simulink model "ConfiguredHevMmVirtualVehicle"  (R2025b)
settings: configuration reference "VehicleVariable" (kept outside this file)
StartFcn:
  | %tic
StopFcn:
  | %toc
model workspace (MAT data in the model file):
  ExtDrvCmdsSwitch : Simulink.Parameter (value not decoded)
  ExtDrvRefSwitch : Simulink.Parameter (value not decoded)
  ExtEnvSwitch : Simulink.Parameter (value not decoded)
  ExtGndSwitch : Simulink.Parameter (value not decoded)
symbols that are objects in the model workspace (value not decoded): ExtDrvCmdsSwitch, ExtDrvRefSwitch, ExtEnvSwitch, ExtGndSwitch
undefined symbols (not defined in the file or in its folder): AmbTemp, BaroPress, CurvGradRef, CurvRef, DCM, DriverAeroRes, DriverDrivelineRes, DriverInitialGear, DriverPreviewDist, DriverRollRes, DriverShiftTime, DriverTimeConst, DriverTractiveForce, EnvAbsPrs, EnvAirTemp, EnvGrvty, EnvNomFrictionScaling, EnvNominalGrade, EnvScnFrictionMap, EnvScnFrictionMapXBpts, EnvScnFrictionMapYBpts, EnvScnHeightMap, EnvScnHeightMapXBpts, EnvScnHeightMapYBpts, EnvWindVelX, EnvWindVelY, EnvWindVelZ, Gnd, Grade, HazzardCmd, HighBeamCmd, lambda_mux, LeftSignalCmd, LngRef, LowBeamCmd, LtrRef, PhiRef, PlntVehDstCGFrntAxl, PlntVehDstCGRearAxl, PlntVehInitLatPos, PlntVehInitLongPos, PlntVehInitPitchAng, PlntVehInitRollAng, PlntVehInitVertPos, PlntVehInitYawAng, PlntVehMass, PlntVehTrckWdth, PlntVehYawMomentInertia, PlntWhlLdRadiusFrnt, PlntWhlLdRadiusRear, RightSignalCmd, ScnCRRadius, Sim3dSensor, Wind, XRef, YRef, Z
libraries: simulink x28, autolibutils x8, autolibsharedcommon x7, vehdynlibscenariocommon x7, vehdynlibviscommon x4, vehdynlibdriver x2, sim3dgroundtruthsensorlib x2, sim3dlib x2, autolibshared x2, sim3dautolib x2, sl3dlib x1, sharedtransform x1
(part 3 of 6)

== system ConfiguredHevMmVirtualVehicle/Driver Commands/Driver Commands/Longitudinal Driver ==
  VehRef : Inport
  VehFdbk : Inport  Port=2
  Env : Inport  Port=3
  Bus Creator1 : BusCreator  Inputs=6
  Bus Selector1 : BusSelector  OutputSignals=DrvCmd.SteerCmd.SteerCmd,DrvRef.LngRef,DrvCmd.AccelCmd.EnblAccelCmd,DrvCmd.AccelCmd.AccelCmd,DrvCmd.AccelCmd.AccelHld,DrvCmd.AccelCmd.AccelZero,DrvCmd.DecelCmd.EnblDecelCmd,DrvCmd.DecelCmd.DecelCmd,DrvCmd.DecelCmd.DecelHld,DrvCmd.DecelCmd.DecelZero
  Constant : Constant  Value=false
  Hill Hold & Stop : Subsystem
  Longitudinal Driver : Subsystem  SystemSampleTime=.01  mask(Longitudinal Driver){extAccelOvr=on, extDecelOvr=on, extAccelHld=on, extDecelHld=on, extAccelZero=on, extDecelZero=on, cntrlType=Predictive, shftType=Reverse, Neutral, Drive, velUnits=m/s, gearOut=on, Kp=10, Ki=5, Kff=.1, Kg=0, VehVelVec=[0 100], KffVec=[.1 .1], KpVec=[10 10], KiVec=[5 5], KgVec=[0 0], m=PlntVehMass, Kpt=DriverTractiveForce, tau=DriverTimeConst, L=DriverPreviewDist, aR=DriverRollRes, bR=DriverDrivelineRes, cR=DriverAeroRes, g=EnvGrvty, vnom=5, Kaw=1, tauerr=.01, tauPt=2, GearInit=DriverInitialGear, tShift=DriverShiftTime, pdlVec=[0.1 0.4 0.5 0.9], upShftTbl=[-1 12.9375 26.4375 39.9375 51.18749999999999 62.4375 72.84375 83.25;-1 16.3125 29.8125 43.3125 54.5624 65.8125 76.78125 87.75;-1 19.6875 33.1875 46.68749999999999 57.9375 69.1875 80.71875 92.25;-1 33 52.5 77.25 100.5 138.75 161.875 185], dwnShftTbl=[1 9.5625 23.0625 36.5625 47.8125 59.0625 68.90625 78.75;1 12.9375 26.4375 39.9375 51.18749999999999 62.4375 72.84375 83.25;1 16.3125 29.8125 43.3125 54.562499 65.8125 76.78125 87.75;1 19.6875 33.1875 46.68749999999999 57.9375 69.1875 80.71875 92.25], tClutch=.5, tRev=.5, tPark=120, aMode=6, UpGearVec=[0  1  2  3  4  5  6  7], DownGearVec=[1  2  3  4  5  6  7  8]}
      mask prompts: extAccelOvr "autoblks_shared:autoblkLongitudinalDriver:blkPrm_extAccelOvr"; extDecelOvr "autoblks_shared:autoblkLongitudinalDriver:blkPrm_extDeccelOvr"; extAccelHld "autoblks_shared:autoblkLongitudinalDriver:blkPrm_extAccelHld"; extDecelHld "autoblks_shared:autoblkLongitudinalDriver:blkPrm_extDeccelHld"; extAccelZero "autoblks_shared:autoblkLongitudinalDriver:blkPrm_extAccelZero"; extDecelZero "autoblks_shared:autoblkLongitudinalDriver:blkPrm_extDeccelZero"; cntrlType "autoblks_shared:autoblkLongitudinalDriver:blkPrm_cntrlType"; shftType "autoblks_shared:autoblkLongitudinalDriver:blkPrm_shftType"; velUnits "autoblks_shared:autoblkLongitudinalDriver:blkPrm_velUnits"; gearOut "autoblks_shared:autoblkLongitudinalDriver:blkPrm_gearOut"; Kp "autoblks_shared:autoblkLongitudinalDriver:blkPrm_Kp"; Ki "autoblks_shared:autoblkLongitudinalDriver:blkPrm_Ki"; Kff "autoblks_shared:autoblkLongitudinalDriver:blkPrm_Kff"; Kg "autoblks_shared:autoblkLongitudinalDriver:blkPrm_Kg"; VehVelVec "autoblks_shared:autoblkLongitudinalDriver:blkPrm_VehVelVec"; KffVec "autoblks_shared:autoblkLongitudinalDriver:blkPrm_KffVec"; KpVec "autoblks_shared:autoblkLongitudinalDriver:blkPrm_KpVec"; KiVec "autoblks_shared:autoblkLongitudinalDriver:blkPrm_KiVec"; KgVec "autoblks_shared:autoblkLongitudinalDriver:blkPrm_KgVec"; m "autoblks_shared:autoblkLongitudinalDriver:blkPrm_m"; Kpt "autoblks_shared:autoblkLongitudinalDriver:blkPrm_Kpt"; tau "autoblks_shared:autoblkLongitudinalDriver:blkPrm_tau"; L "autoblks_shared:autoblkLongitudinalDriver:blkPrm_L"; aR "autoblks_shared:autoblkLongitudinalDriver:blkPrm_aR"; bR "autoblks_shared:autoblkLongitudinalDriver:blkPrm_bR"; cR "autoblks_shared:autoblkLongitudinalDriver:blkPrm_cR"; g "autoblks_shared:autoblkLongitudinalDriver:blkPrm_g"; vnom "autoblks_shared:autoblkLongitudinalDriver:blkPrm_vnom"; Kaw "autoblks_shared:autoblkLongitudinalDriver:blkPrm_Kaw"; tauerr "autoblks_shared:autoblkLongitudinalDriver:blkPrm_tauerr"; tauPt "autoblks_shared:autoblkLongitudinalDriver:blkPrm_tauPt"; GearInit "autoblks_shared:autoblkLongitudinalDriver:blkPrm_GearInit"; tShift "autoblks_shared:autoblkLongitudinalDriver:blkPrm_tShift"; pdlVec "autoblks_shared:autoblkLongitudinalDriver:blkPrm_pdlVec"; upShftTbl "autoblks_shared:autoblkLongitudinalDriver:blkPrm_upShftTbl"; dwnShftTbl "autoblks_shared:autoblkLongitudinalDriver:blkPrm_dwnShftTbl"; tClutch "autoblks_shared:autoblkLongitudinalDriver:blkPrm_tClutch"; tRev "autoblks_shared:autoblkLongitudinalDriver:blkPrm_tRev"; tPark "autoblks_shared:autoblkLongitudinalDriver:blkPrm_tPark"; UpGearVec "autoblks_shared:autoblkLongitudinalDriver:blkPrm_UpGearVec"; DownGearVec "autoblks_shared:autoblkLongitudinalDriver:blkPrm_DownGearVec"
      mask help: autoblks_shared:autoblkLongitudinalDriver:blkDesc
      mask init:
      | [~]=autosharedicon('autoliboperlong',gcb,0);
      mask Help: eval('autosharedhelp(''pbopmodlong'')');
      mask TypeOptions cntrlType: autoblks_shared:autoblkLongitudinalDriver:blkCmb_cntrlType_c1 | autoblks_shared:autoblkLongitudinalDriver:blkCmb_cntrlType_c2 | autoblks_shared:autoblkLongitudinalDriver:blkCmb_cntrlType_c3
      mask Callback cntrlType: [~]=autosharedicon('autoliboperlong',gcb,1);
      mask TypeOptions shftType: Longitudinal Driver/shftType
      mask Callback shftType: [~]=autosharedicon('autoliboperlong',gcb,1);
      mask TypeOptions velUnits: VelRef/Unit
      mask Callback velUnits: [~]=autosharedicon('autoliboperlong',gcb,1);
      mask DialogControl modeConfig Prompt: autoblks_shared:autoblkLongitudinalDriver:blkDlg_modeConfig
      mask DialogControl sigConfigPanel Prompt: autoblks_shared:autoblkLongitudinalDriver:blkDlg_sigConfigPanel
      mask DialogControl extAccelOvr Prompt: Accelerator override
      mask DialogControl extDecelOvr Prompt: Decelerator override
      mask DialogControl extAccelHld Prompt: Accelerator hold
      mask DialogControl extDecelHld Prompt: Decelerator hold
      mask DialogControl extAccelZero Prompt: Accelerator disable
      mask DialogControl extDecelZero Prompt: Decelerator disable
      mask DialogControl cntrlType Prompt: Control type, cntrlType:
      mask DialogControl shftType Prompt: Shift type, shftType:
      mask DialogControl velUnits Prompt: Reference and feedback units, velUnits [velUnits]:
      mask DialogControl gearOut Prompt: Output gear signal
      mask DialogControl CntrlParamPanel Prompt: autoblks_shared:autoblkLongitudinalDriver:blkDlg_CntrlParamPanel
      mask DialogControl PIParam Prompt: autoblks_shared:autoblkLongitudinalDriver:blkDlg_PIParam
      mask DialogControl Kp Prompt: Proportional gain, Kp []:
      mask DialogControl Ki Prompt: Integral gain, Ki []:
      mask DialogControl Kff Prompt: Velocity feed-forward, Kff []:
      mask DialogControl Kg Prompt: Grade angle feed-forward, Kg [1/deg]:
      mask DialogControl PISchedParam Prompt: autoblks_shared:autoblkLongitudinalDriver:blkDlg_PISchedParam
      mask DialogControl VehVelVec Prompt: Velocity gain breakpoints:
      mask DialogControl KffVec Prompt: Velocity feed-forward gain values, KffVec []:
      mask DialogControl KpVec Prompt: Proportional gain values, KpVec []:
      mask DialogControl KiVec Prompt: Integral gain values, KiVec []:
      mask DialogControl KgVec Prompt: Grade angle feed-forward values, KgVec [1/deg]:
      mask DialogControl PredParam Prompt: autoblks_shared:autoblkLongitudinalDriver:blkDlg_PredParam
      mask DialogControl m Prompt: Vehicle mass, m [kg]:
      mask DialogControl Kpt Prompt: Effective vehicle total tractive force, Kpt [N]:
      mask DialogControl tau Prompt: Driver response time, tau [s]:
      mask DialogControl L Prompt: Preview distance, L [m]:
      mask DialogControl aR Prompt: Rolling resistance coefficient, aR [N]:
      mask DialogControl bR Prompt: Rolling and driveline resistance coefficient, bR [N*s/m]:
      mask DialogControl cR Prompt: Aerodynamic drag coefficient, cR [N*s^2/m^2]:
      mask DialogControl g Prompt: Gravitational constant, g [m/s^2]:
      mask DialogControl vnom Prompt: Nominal speed, vnom [velUnits]:
      mask DialogControl Kaw Prompt: Anti-windup, Kaw []:
      mask DialogControl tauerr Prompt: Error filter time constant, tauerr [s]:
      mask DialogControl tauPt Prompt: Powertrain time constant, tauPt [s]:
      mask DialogControl shiftParamPanel Prompt: autoblks_shared:autoblkLongitudinalDriver:blkDlg_shiftParamPanel
      mask DialogControl GearInit Prompt: Initial gear, GearInit []:
      mask DialogControl tShift Prompt: Time required to shift, tShift [s]:
      mask DialogControl pdlVec Prompt: Up and down shift accelerator pedal positions, pdlVec []:
      mask DialogControl upShftTbl Prompt: Upshift velocity data table, upShftTbl [velUnits]:
      mask DialogControl dwnShftTbl Prompt: Downshift velocity data table, dwnShftTbl [velUnits]:
      mask DialogControl tClutch Prompt: Time required to shift, tClutch [s]:
      mask DialogControl tRev Prompt: Time required to engage reverse from neutral, tRev [s]:
      mask DialogControl tPark Prompt: Time required to engage park from neutral, tPark [s]:
      mask DialogControl UpGearVec Prompt: Upshift gear vector, UpGearVec []:
      mask DialogControl DownGearVec Prompt: Downshift gear vector, DownGearVec []:
      mask Display:
      | try
      |     IconInfo = autosharedicon('autoliboperlong', gcb, 4);
      | 
      |     image(IconInfo.image, IconInfo.position);
      | 
      |     for i = 1:numel(IconInfo.lconn)
      |         port_label('lconn', i, IconInfo.lconn{i})
      |     end
      | 
      |     for j = 1:numel(IconInfo.rconn)
      |         port_label('rconn', j, IconInfo.rconn{j})
      |     end
      | 
      |     for k = 1:numel(IconInfo.input)
      |         port_label('input', k, IconInfo.input{k})
      |     end
      | 
      |     for m = 1:numel(IconInfo.output)
      |         port_label('output', m, IconInfo.output{m})
      |     end
      | catch
      |     fprintf('Longitudinal \n Driver')
      | end
  Signal Specification : SignalSpecification  Unit=rad
  Terminator3 : Terminator
  To Nonvirtual Bus : SignalConversion  ConversionOutput=Virtual bus  OverrideOpt=off
  Unit Conversion : UnitConversion
  Unit Conversion1 : UnitConversion
  VVCLightsCmd : Constant  Value=0  OutDataTypeStr=Bus: VVCLightsCmdBUS  SampleTime=-1
  Driver : Outport  VectorParamsAs1DForOutWhenUnconnected=off
  wires:
  Signal Specification/1 -> Bus Creator1/1  "SteerCmd"
  To Nonvirtual Bus/1 -> Bus Creator1/6  "LightsCmd"
  VVCLightsCmd/1 -> To Nonvirtual Bus/1
  Hill Hold & Stop/6(Grade) -> Longitudinal Driver/11(Grade)
  Hill Hold & Stop/5(VelFdbk) -> Longitudinal Driver/10(VelFdbk)
  Bus Selector1/5 -> Longitudinal Driver/4(AccelHld)  "<AccelHld>"
  Unit Conversion1/1 -> Longitudinal Driver/1(VelRef), Hill Hold & Stop/1(LngRef)
  Hill Hold & Stop/4(DecelZero) -> Longitudinal Driver/9(DecelZero)
  Hill Hold & Stop/3(DecelHld) -> Longitudinal Driver/8(DecelHld)
  Env/1 -> Hill Hold & Stop/6(Env)
  Hill Hold & Stop/1(EnblDecelOvr) -> Longitudinal Driver/6(EnblDecelOvr)
  Hill Hold & Stop/2(DecelOvrCmd) -> Longitudinal Driver/7(DecelOvrCmd)
  Bus Selector1/10 -> Hill Hold & Stop/5(<DecelZero>)  "<DecelZero>"
  Bus Selector1/9 -> Hill Hold & Stop/4(<DecelHld>)  "<DecelHld>"
  Bus Selector1/8 -> Hill Hold & Stop/3(<DecelOvrCmd>)  "<DecelCmd>"
  Bus Selector1/7 -> Hill Hold & Stop/2(<EnblDecelCmd>)  "<EnblDecelCmd>"
  Bus Selector1/6 -> Longitudinal Driver/5(AccelZero)  "<AccelZero>"
  Bus Selector1/4 -> Longitudinal Driver/3(AccelOvrCmd)  "<AccelCmd>"
  Bus Selector1/3 -> Longitudinal Driver/2(EnblAccelOvr)  "<EnblAccelCmd>"
  Constant/1 -> Bus Creator1/5  "IgnSwtch"
  Bus Selector1/1 -> Unit Conversion/1  "<SteerCmd>"
  Longitudinal Driver/4(GearCmd) -> Bus Creator1/4  "GearCmd"
  Longitudinal Driver/2(AccelCmd) -> Bus Creator1/2  "AccelCmd"
  VehFdbk/1 -> Hill Hold & Stop/7(VehFdbk)
  VehRef/1 -> Bus Selector1/1
  Bus Selector1/2 -> Unit Conversion1/1  "<LngRef>"
  Longitudinal Driver/1(Info) -> Terminator3/1
  Longitudinal Driver/3(DecelCmd) -> Bus Creator1/3  "DecelCmd"
  Unit Conversion/1 -> Signal Specification/1
  Bus Creator1/1 -> Driver/1

== system ConfiguredHevMmVirtualVehicle/Driver Commands/Driver Commands/No Driver ==
  VehRef : Inport
  VehFdbk : Inport  Port=2
  Env : Inport  Port=3
  Bus Creator1 : BusCreator  Inputs=6
  Bus Selector1 : BusSelector  OutputSignals=DrvCmd.SteerCmd.SteerCmd,DrvCmd.AccelCmd.AccelCmd,DrvCmd.DecelCmd.DecelCmd,DrvCmd.TransCmd.GearCmd,DrvCmd.IgnModeCmd,DrvCmd.LightsCmd
  Data Type Conversion : DataTypeConversion  SaturateOnIntegerOverflow=off  RndMeth=Floor
  Data Type Conversion1 : DataTypeConversion  SaturateOnIntegerOverflow=off  RndMeth=Floor
  Signal Specification{,1..3} (4 alike) : SignalSpecification  Unit=1
  Signal Specification4 : SignalSpecification  Unit=rad
  Terminator : Terminator
  Terminator1 : Terminator
  To Nonvirtual Bus : SignalConversion  ConversionOutput=Virtual bus  OverrideOpt=off
  Unit Conversion{,1..3} (4 alike) : UnitConversion
  Driver : Outport  VectorParamsAs1DForOutWhenUnconnected=off
  wires:
  Unit Conversion/1 -> Signal Specification4/1
  Data Type Conversion/1 -> Signal Specification3/1
  Unit Conversion3/1 -> Signal Specification2/1
  Unit Conversion2/1 -> Signal Specification1/1
  Unit Conversion1/1 -> Signal Specification/1
  Data Type Conversion1/1 -> Unit Conversion3/1
  Bus Selector1/5 -> Data Type Conversion/1  "<IgnModeCmd>"
  Bus Selector1/6 -> To Nonvirtual Bus/1  "<LightsCmd>"
  Bus Selector1/4 -> Data Type Conversion1/1  "<GearCmd>"
  Bus Selector1/3 -> Unit Conversion2/1  "<DecelCmd>"
  To Nonvirtual Bus/1 -> Bus Creator1/6  "LightsCmd"
  Env/1 -> Terminator1/1
  Signal Specification3/1 -> Bus Creator1/5  "IgnSwtch"
  Bus Selector1/1 -> Unit Conversion/1  "<SteerCmd>"
  Signal Specification2/1 -> Bus Creator1/4  "GearCmd"
  Signal Specification/1 -> Bus Creator1/2  "AccelCmd"
  VehFdbk/1 -> Terminator/1
  VehRef/1 -> Bus Selector1/1
  Bus Selector1/2 -> Unit Conversion1/1  "<AccelCmd>"
  Signal Specification1/1 -> Bus Creator1/3  "DecelCmd"
  Signal Specification4/1 -> Bus Creator1/1  "SteerCmd"
  Bus Creator1/1 -> Driver/1

== system ConfiguredHevMmVirtualVehicle/Driver Commands/Driver Commands/Open Loop ==
  VehFdbk : Inport
  SteerCmd : Inport  Port=2
  AccelCmd : Inport  Port=3
  BrakeCmd : Inport  Port=4
  GearCmd : Inport  Port=5
  Bus Creator1 : BusCreator  Inputs=6
  Constant : Constant  Value=false
  Signal Specification : SignalSpecification  Unit=1
  Signal Specification1 : SignalSpecification  Unit=1
  Signal Specification2 : SignalSpecification  Unit=1
  Terminator : Terminator
  To Nonvirtual Bus : SignalConversion  ConversionOutput=Virtual bus  OverrideOpt=off
  Unit Conversion : UnitConversion
  VVCLightsCmd : Constant  Value=0  OutDataTypeStr=Bus: VVCLightsCmdBUS  SampleTime=-1
  Wheel Angle Limit * Steer Ratio : Gain  Gain=40*pi/180*18
  Driver : Outport  VectorParamsAs1DForOutWhenUnconnected=off
  wires:
  To Nonvirtual Bus/1 -> Bus Creator1/6  "LightsCmd"
  VVCLightsCmd/1 -> To Nonvirtual Bus/1
  Constant/1 -> Bus Creator1/5  "IgnSwtch"
  Signal Specification1/1 -> Bus Creator1/3  "DecelCmd"
  GearCmd/1 -> Signal Specification2/1
  Signal Specification/1 -> Bus Creator1/2  "AccelCmd"
  SteerCmd/1 -> Unit Conversion/1
  VehFdbk/1 -> Terminator/1
  AccelCmd/1 -> Signal Specification/1
  Unit Conversion/1 -> Wheel Angle Limit * Steer Ratio/1
  Bus Creator1/1 -> Driver/1
  Wheel Angle Limit * Steer Ratio/1 -> Bus Creator1/1  "SteerCmd"
  BrakeCmd/1 -> Signal Specification1/1
  Signal Specification2/1 -> Bus Creator1/4  "GearCmd"

== system ConfiguredHevMmVirtualVehicle/Driver Commands/Driver Commands/Predictive Driver ==
  VehRef : Inport
  VehFdbk : Inport  Port=2
  Env : Inport  Port=3
  Bus Creator1 : BusCreator  Inputs=6
  Bus Selector : BusSelector  OutputSignals=Body.InertFrm.Cg.Disp.Y,Body.InertFrm.Cg.Vel.Ydot,Body.InertFrm.Cg.Ang.psi,Body.BdyFrm.Cg.AngVel.r
  Bus Selector1 : BusSelector  OutputSignals=DrvRef.LngRef,DrvRef.LtrRef,DrvCmd.SteerCmd.EnblSteerCmd,DrvCmd.SteerCmd.SteerCmd,DrvCmd.SteerCmd.SteerHld,DrvCmd.SteerCmd.SteerZero,DrvCmd.AccelCmd.EnblAccelCmd,DrvCmd.AccelCmd.AccelCmd,DrvCmd.AccelCmd.AccelHld,DrvCmd.AccelCmd.AccelZero,DrvCmd.DecelCmd.EnblDecelCmd,DrvCmd.DecelCmd.DecelCmd,DrvCmd.DecelCmd.DecelHld,DrvCmd.DecelCmd.DecelZero
  Constant : Constant  Value=false
  Hill Hold & Stop : Subsystem
  Linear Predictive Driver : vehdynlibdriver/Predictive Driver  extAccelOvr=on  extDecelOvr=on  extAccelHld=on  extDecelHld=on  extAccelZero=on  extDecelZero=on  extSteerOvr=on  extSteerHld=on  extSteerZero=on  cntrlType=Predictive  cntrlTypeLat=Predictive  shftType=Reverse, Neutral, Drive  coordMode=SAE J670 (Z-down)  refType=Reference pose  velUnits=m/s  angUnits=rad  gearOut=on  steerOut=on  Kp=3  Ki=1  Kff=1  Kg=0  VehVelVec=[0 100]  KffVec=[.1 .1]  KpVec=[10 10]  KiVec=[5 5]  KgVec=[0 0]  vnom=5  Kaw=1  tauerr=.075  tau=DriverTimeConst  L=DriverPreviewDist  Kpt=DriverTractiveForce  aR=DriverRollRes  bR=DriverDrivelineRes  cR=DriverAeroRes  g=EnvGrvty  vecPose=off  dynamMode=off  PositionGainF=2.5  PositionGainR=2.5  YawRateGain=.2  DelayGain=.2  enableDrift=off  BetaRef=10  KpBeta=1  KpDrift=1  KdDrift=1  KpPsi=1  KOmega=.1  tOmega=.1  a=PlntVehDstCGFrntAxl  b=PlntVehDstCGRearAxl  m=PlntVehMass  Cy_f=DriverFrontCornerStiff  Cy_r=DriverRearCornerStiff  I=PlntVehYawMomentInertia  Ksteer=PlntSteerRatio  theta=DriverWheelRange  Idl=1  Re=PlntWhlLdRadius  lambda_mu=1  GearInit=DriverInitialGear  tShift=DriverShiftTime  pdlVec=[0.1 0.4 0.5 0.9]  upShftTbl=[-1 12.9375 26.4375 39.9375 51.18749999999999 62.4375 72.84375 83.25;-1 16.3125 29.8125 43.3125 54.5624 65.8125 76.78125 87.75;-1 19.6875 33.1875 46.68749999999999 57.9375 69.1875 80.71875 92.25;-1 33 52.5 77.25 100.5 138.75 161.875 185]  dwnShftTbl=[-1 12.9375 26.4375 39.9375 51.18749999999999 62.4375 72.84375 83.25;-1 16.3125 29.8125 43.3125 54.5624 65.8125 76.78125 87.75;-1 19.6875 33.1875 46.68749999999999 57.9375 69.1875 80.71875 92.25;-1 33 52.5 77.25 100.5 138.75 161.875 185]  tClutch=.5  tRev=.5  tPark=120  UpGearVec="[0  1  2  3  4  5  6  7]"  DownGearVec="[1  2  3  4  5  6  7  8]"  aMode=2
  Terminator : Terminator
  To Nonvirtual Bus : SignalConversion  ConversionOutput=Virtual bus  OverrideOpt=off
  Unit Conversion : UnitConversion
  VVCLightsCmd : Constant  Value=0  OutDataTypeStr=Bus: VVCLightsCmdBUS  SampleTime=-1
  Driver : Outport  VectorParamsAs1DForOutWhenUnconnected=off
  wires:
  Bus Selector1/14 -> Hill Hold & Stop/5(<DecelZero>)  "<DecelZero>"
  To Nonvirtual Bus/1 -> Bus Creator1/6  "LightsCmd"
  VVCLightsCmd/1 -> To Nonvirtual Bus/1
  Unit Conversion/1 -> Linear Predictive Driver/1, Hill Hold & Stop/1(LngRef)
  Hill Hold & Stop/1(EnblDecelOvr) -> Linear Predictive Driver/11
  Hill Hold & Stop/2(DecelOvrCmd) -> Linear Predictive Driver/12
  Hill Hold & Stop/3(DecelHld) -> Linear Predictive Driver/13
  Hill Hold & Stop/4(DecelZero) -> Linear Predictive Driver/14
  Hill Hold & Stop/6(VelFdbk) -> Linear Predictive Driver/16
  Hill Hold & Stop/5(Grade) -> Linear Predictive Driver/15
  Env/1 -> Hill Hold & Stop/6(Env)
  Bus Selector1/13 -> Hill Hold & Stop/4(<DecelHld>)  "<DecelHld>"
  Bus Selector1/12 -> Hill Hold & Stop/3(<DecelOvrCmd>)  "<DecelCmd>"
  Bus Selector1/11 -> Hill Hold & Stop/2(<EnblDecelCmd>)  "<EnblDecelCmd>"
  Bus Selector1/9 -> Linear Predictive Driver/9  "<AccelHld>"
  Bus Selector1/8 -> Linear Predictive Driver/8  "<AccelCmd>"
  Bus Selector1/7 -> Linear Predictive Driver/7  "<EnblAccelCmd>"
  Bus Selector1/6 -> Linear Predictive Driver/6  "<SteerZero>"
  Bus Selector1/5 -> Linear Predictive Driver/5  "<SteerHld>"
  Bus Selector1/4 -> Linear Predictive Driver/4  "<SteerCmd>"
  Bus Selector1/3 -> Linear Predictive Driver/3  "<EnblSteerCmd>"
  Constant/1 -> Bus Creator1/5  "IgnSwtch"
  Linear Predictive Driver/5 -> Bus Creator1/4  "GearCmd"
  Linear Predictive Driver/4 -> Bus Creator1/3  "DecelCmd"
  Linear Predictive Driver/2 -> Bus Creator1/1  "SteerCmd"
  Bus Selector1/1 -> Unit Conversion/1  "<LngRef>"
  VehRef/1 -> Bus Selector1/1
  Bus Selector/4 -> Linear Predictive Driver/20  "<r>"
  Bus Selector1/2 -> Linear Predictive Driver/2  "<LtrRef>"
  VehFdbk/1 -> Bus Selector/1, Hill Hold & Stop/7(VehFdbk)
  Bus Selector/3 -> Linear Predictive Driver/19  "<psi>"
  Linear Predictive Driver/1 -> Terminator/1
  Bus Creator1/1 -> Driver/1
  Bus Selector1/10 -> Linear Predictive Driver/10  "<AccelZero>"
  Bus Selector/1 -> Linear Predictive Driver/17  "<Y>"
  Linear Predictive Driver/3 -> Bus Creator1/2  "AccelCmd"
  Bus Selector/2 -> Linear Predictive Driver/18  "<Ydot>"

== system ConfiguredHevMmVirtualVehicle/Driver Commands/Driver Commands/Predictive Stanley Driver ==
  VehRef : Inport
  VehFdbk : Inport  Port=2
  Env : Inport  Port=3
  Bus Creator1 : BusCreator  Inputs=6
  Bus Selector : BusSelector  OutputSignals=Body.InertFrm.Cg.Disp.X,Body.InertFrm.Cg.Disp.Y,Body.InertFrm.Cg.Ang.psi,Body.BdyFrm.Cg.AngVel.r
  Bus Selector1 : BusSelector  OutputSignals=DrvRef.LngRef,DrvRef.XRef,DrvRef.YRef,DrvRef.PhiRef,DrvCmd.SteerCmd.EnblSteerCmd,DrvCmd.SteerCmd.SteerCmd,DrvCmd.SteerCmd.SteerHld,DrvCmd.SteerCmd.SteerZero,DrvCmd.AccelCmd.EnblAccelCmd,DrvCmd.AccelCmd.AccelCmd,DrvCmd.AccelCmd.AccelHld,DrvCmd.AccelCmd.AccelZero,DrvCmd.DecelCmd.EnblDecelCmd,DrvCmd.DecelCmd.DecelCmd,DrvCmd.DecelCmd.DecelHld,DrvCmd.DecelCmd.DecelZero,DrvRef.CurvRef
  Constant : Constant  Value=false
  Hill Hold & Stop : Subsystem
  Linear Predictive Driver : vehdynlibdriver/Predictive Driver  extAccelOvr=on  extDecelOvr=on  extAccelHld=on  extDecelHld=on  extAccelZero=on  extDecelZero=on  extSteerOvr=on  extSteerHld=on  extSteerZero=on  cntrlType=Predictive  cntrlTypeLat=Stanley  shftType=Reverse, Neutral, Drive  coordMode=SAE J670 (Z-down)  refType=Reference pose  velUnits=m/s  angUnits=rad  gearOut=on  steerOut=on  Kp=3  Ki=1  Kff=1  Kg=0  VehVelVec=[0 100]  KffVec=[.1 .1]  KpVec=[10 10]  KiVec=[5 5]  KgVec=[0 0]  vnom=5  Kaw=1  tauerr=.075  tau=DriverTimeConst  L=DriverPreviewDist  Kpt=DriverTractiveForce  aR=DriverRollRes  bR=DriverDrivelineRes  cR=DriverAeroRes  g=EnvGrvty  vecPose=off  dynamMode=on  PositionGainF=DriverPositionGainF  PositionGainR=DriverPositionGainR  YawRateGain=DriverYawRateGain  DelayGain=DriverDelayGain  enableDrift=off  BetaRef=10  KpBeta=1  KpDrift=1  KdDrift=1  KpPsi=1  KOmega=.1  tOmega=.1  a=PlntVehDstCGFrntAxl  b=PlntVehDstCGRearAxl  m=PlntVehMass  Cy_f=DriverFrontCornerStiff  Cy_r=DriverRearCornerStiff  I=PlntVehYawMomentInertia  Ksteer=PlntSteerRatio  theta=DriverWheelRange  Idl=1  Re=PlntWhlLdRadius  lambda_mu=1  GearInit=DriverInitialGear  tShift=DriverShiftTime  pdlVec=[0.1 0.4 0.5 0.9]  upShftTbl=[-1 12.9375 26.4375 39.9375 51.18749999999999 62.4375 72.84375 83.25;-1 16.3125 29.8125 43.3125 54.5624 65.8125 76.78125 87.75;-1 19.6875 33.1875 46.68749999999999 57.9375 69.1875 80.71875 92.25;-1 33 52.5 77.25 100.5 138.75 161.875 185]  dwnShftTbl=[-1 12.9375 26.4375 39.9375 51.18749999999999 62.4375 72.84375 83.25;-1 16.3125 29.8125 43.3125 54.5624 65.8125 76.78125 87.75;-1 19.6875 33.1875 46.68749999999999 57.9375 69.1875 80.71875 92.25;-1 33 52.5 77.25 100.5 138.75 161.875 185]  tClutch=.5  tRev=.5  tPark=120  UpGearVec="[0  1  2  3  4  5  6  7]"  DownGearVec="[1  2  3  4  5  6  7  8]"  aMode=2
  Terminator : Terminator
  To Nonvirtual Bus : SignalConversion  ConversionOutput=Virtual bus  OverrideOpt=off
  Unit Conversion : UnitConversion
  VVCLightsCmd : Constant  Value=0  OutDataTypeStr=Bus: VVCLightsCmdBUS  SampleTime=-1
  Driver : Outport  VectorParamsAs1DForOutWhenUnconnected=off
  wires:
  Bus Selector1/13 -> Hill Hold & Stop/2(<EnblDecelCmd>)  "<EnblDecelCmd>"
  Bus Selector1/14 -> Hill Hold & Stop/3(<DecelOvrCmd>)  "<DecelCmd>"
  Bus Selector1/15 -> Hill Hold & Stop/4(<DecelHld>)  "<DecelHld>"
  Bus Selector1/16 -> Hill Hold & Stop/5(<DecelZero>)  "<DecelZero>"
  Bus Selector1/17 -> Hill Hold & Stop/6(<CurvRef>)  "<CurvRef>"
  Bus Selector1/12 -> Linear Predictive Driver/12  "<AccelZero>"
  Bus Selector/1 -> Linear Predictive Driver/20  "<X>"
  Bus Selector/2 -> Linear Predictive Driver/21  "<Y>"
  Bus Selector/3 -> Linear Predictive Driver/22  "<psi>"
  Bus Selector1/2 -> Linear Predictive Driver/2  "<XRef>"
  Bus Selector1/3 -> Linear Predictive Driver/3  "<YRef>"
  Bus Selector1/4 -> Linear Predictive Driver/4  "<PhiRef>"
  Bus Selector1/5 -> Linear Predictive Driver/5  "<EnblSteerCmd>"
  Bus Selector1/10 -> Linear Predictive Driver/10  "<AccelCmd>"
  Bus Selector1/6 -> Linear Predictive Driver/6  "<SteerCmd>"
  Bus Selector1/9 -> Linear Predictive Driver/9  "<EnblAccelCmd>"
  Bus Selector1/7 -> Linear Predictive Driver/7  "<SteerHld>"
  Bus Selector1/8 -> Linear Predictive Driver/8  "<SteerZero>"
  To Nonvirtual Bus/1 -> Bus Creator1/6  "LightsCmd"
  VVCLightsCmd/1 -> To Nonvirtual Bus/1
  Hill Hold & Stop/6(CurvRef) -> Linear Predictive Driver/18
  Hill Hold & Stop/5(Grade) -> Linear Predictive Driver/17
  Bus Selector/4 -> Linear Predictive Driver/23  "<r>"
  Linear Predictive Driver/3 -> Bus Creator1/2  "AccelCmd"
  Bus Creator1/1 -> Driver/1
  Linear Predictive Driver/1 -> Terminator/1
  VehFdbk/1 -> Bus Selector/1, Hill Hold & Stop/8(VehFdbk)
  VehRef/1 -> Bus Selector1/1
  Bus Selector1/1 -> Unit Conversion/1  "<LngRef>"
  Linear Predictive Driver/2 -> Bus Creator1/1  "SteerCmd"
  Linear Predictive Driver/4 -> Bus Creator1/3  "DecelCmd"
  Linear Predictive Driver/5 -> Bus Creator1/4  "GearCmd"
  Constant/1 -> Bus Creator1/5  "IgnSwtch"
  Bus Selector1/11 -> Linear Predictive Driver/11  "<AccelHld>"
  Env/1 -> Hill Hold & Stop/7(Env)
  Hill Hold & Stop/7(VelFdbk) -> Linear Predictive Driver/19
  Hill Hold & Stop/4(DecelZero) -> Linear Predictive Driver/16
  Hill Hold & Stop/3(DecelHld) -> Linear Predictive Driver/15
  Hill Hold & Stop/2(DecelOvrCmd) -> Linear Predictive Driver/14
  Hill Hold & Stop/1(EnblDecelOvr) -> Linear Predictive Driver/13
  Unit Conversion/1 -> Linear Predictive Driver/1, Hill Hold & Stop/1(LngRef)

== system ConfiguredHevMmVirtualVehicle/Environment/Ground Feedback/3D Engine ==
  WheelFdbk : Inport
  3D Engine Source : Subsystem  Variant=on  VariantControl=Choice  mask(Terrain Source){terrType=Single point}
      mask prompts: terrType "Terrain feedback type:"
      mask help:
      | This variant subsystem provides the option for:
      | - a single point of contact for each wheel with minimal post-processing ideal for smooth surfaces and maximum run-time performance.
      | - multiple points of contact per wheel which may be used when interested in non-smooth terrain at a higher computational cost and requires Vehicle Dynamics Blockset.
      mask TypeOptions terrType: Single point | Multiple points
  Z : Outport  VectorParamsAs1DForOutWhenUnconnected=off
  DCM : Outport  Port=2  VectorParamsAs1DForOutWhenUnconnected=off
  wires:
  WheelFdbk/1 -> 3D Engine Source/1(WheelFdbk)
  3D Engine Source/1(z) -> Z/1
  3D Engine Source/2(DCM) -> DCM/1

== system ConfiguredHevMmVirtualVehicle/Environment/Ground Feedback/Constant ==
  Bus Creator : BusCreator  Inputs=4
  Constant1 : Constant  Value=zeros(4,1)
  Constant2 : Constant  Value=repmat(eye(3),1,1,4)  SampleTime=-1
  Demux : Demux
  Signal Specification : SignalSpecification  Unit=m
  Z : Outport  VectorParamsAs1DForOutWhenUnconnected=off
  DCM : Outport  Port=2  VectorParamsAs1DForOutWhenUnconnected=off
  wires:
  Constant1/1 -> Signal Specification/1
  Signal Specification/1 -> Demux/1
  Demux/4 -> Bus Creator/4  "G_RR_z"
  Demux/1 -> Bus Creator/1  "G_FL_z"
  Demux/3 -> Bus Creator/3  "G_RL_z"
  Demux/2 -> Bus Creator/2  "G_FR_z"
  Bus Creator/1 -> Z/1  "z"
  Constant2/1 -> DCM/1  "DCM"

== system ConfiguredHevMmVirtualVehicle/Environment/Ground Feedback/Height Map ==
  InertFrm : Inport
  "2D Lookup Tbl for Elevation, Z" : Subsystem  TreatAsAtomicUnit=on
      mask init:
      | [~]=vehdynicon('vehdynblk',gcb);
  Bus Creator : BusCreator  Inputs=4
  Bus Selector : BusSelector  OutputSignals=FrntAxl.Lft.Disp.X,FrntAxl.Rght.Disp.X,RearAxl.Lft.Disp.X,RearAxl.Rght.Disp.X
  Bus Selector1 : BusSelector  OutputSignals=FrntAxl.Lft.Disp.Y,FrntAxl.Rght.Disp.Y,RearAxl.Lft.Disp.Y,RearAxl.Rght.Disp.Y
  Constant2 : Constant  Value=repmat(eye(3),1,1,4)  SampleTime=-1
  Demux : Demux
  Signal Specification : SignalSpecification  Unit=m
  Wheel Coordinates : Subsystem
  Z : Outport
  DCM : Outport  Port=2
  wires:
  "2D Lookup Tbl for Elevation, Z"/1(Z) -> Signal Specification/1
  Bus Selector1/4 -> Wheel Coordinates/8(RearAxlRghtY)  "<Y>"
  Bus Selector1/3 -> Wheel Coordinates/7(RearAxlLftY)  "<Y>"
  Bus Selector/1 -> Wheel Coordinates/1(FrntAxlLftX)  "<X>"
  Bus Selector/2 -> Wheel Coordinates/2(FrntAxlRghtX)  "<X>"
  Bus Selector1/2 -> Wheel Coordinates/6(FrntAxlRghtY)  "<Y>"
  Bus Selector/4 -> Wheel Coordinates/4(RearAxlRghtX)  "<X>"
  Bus Selector/3 -> Wheel Coordinates/3(RearAxlLftX)  "<X>"
  Bus Selector1/1 -> Wheel Coordinates/5(FrntAxlLftY)  "<Y>"
  Wheel Coordinates/2(YWhl) -> "2D Lookup Tbl for Elevation, Z"/2(YWhl)
  Wheel Coordinates/1(XWhl) -> "2D Lookup Tbl for Elevation, Z"/1(XWhl)
  InertFrm/1 -> Bus Selector1/1, Bus Selector/1
  Demux/2 -> Bus Creator/2  "G_FR_z"
  Demux/1 -> Bus Creator/1  "G_FL_z"
  Demux/4 -> Bus Creator/4  "G_RR_z"
  Demux/3 -> Bus Creator/3  "G_RL_z"
  Bus Creator/1 -> Z/1  "z"
  Signal Specification/1 -> Demux/1
  Constant2/1 -> DCM/1  "DCM"

== system ConfiguredHevMmVirtualVehicle/Environment/Ground Feedback/Ideal Inclined Plane ==
  InertFrm : Inport
  Bus Creator : BusCreator  Inputs=4
  Bus Selector : BusSelector  OutputSignals=FrntAxl.Lft.Disp.X,FrntAxl.Rght.Disp.X,RearAxl.Lft.Disp.X,RearAxl.Rght.Disp.X
  Bus Selector1 : BusSelector  OutputSignals=FrntAxl.Lft.Disp.Y,FrntAxl.Rght.Disp.Y,RearAxl.Lft.Disp.Y,RearAxl.Rght.Disp.Y
  Demux : Demux
  Ideal Inclined Plane : Subsystem  mask(Ideal Plane Elevation Generator){phi_o=0, theta_o=0, Z_o=0, psi_o=-PlntVehInitYawAng, phi_est=0, theta_est=0, Z_est=5, plane3D=off, planeX=200, planeY=200}
      mask prompts: phi_o "Initial plane bank angle (about global X axis) [rad]:"; theta_o "Initial plane pitch angle (about global Y axis)  [rad]:"; Z_o "Initial plane elevation (at [0,0,0]) [m]"; psi_o "Initial vehicle yaw angle (about global Z axis) [rad]:"; phi_est "Estimated initial vehicle roll angle [rad]:"; theta_est "Estimated initial vehicle pitch angle [rad]:"; Z_est "Estimated initial vehicle elevation [m]"; plane3D "Enable 3D visualization of plane. Requires the Simulink 3D Animation and the 3D visualization enabled (in the Visualization subsystem). The Empty Scene is recommended when activated."; planeX "Total plane length (in X dimension) [m]:"; planeY "Total plane width (in Y dimension) [m]:"
      mask help:
      | This block accepts time varying bank and pitch angles for an idealized planar surface centered at the global origin (Z+up).
      | The plane roll or bank angle, phi, is about the X axis and pitch angle, theta (negative grade), is about the Y axis.
      | A static vertical offset, Z_o, is also permited.
      | Based on the initial plane angles and vertical offset and vehicle pose, estimates of the initial vehicle roll and pitch are calculated (in the vehicle Z+ down frame). These values can be optionally used to udpate the sldds.
      | Caution should be used to esnure the input signals and initial parameters are consistent at initialzation time.
      | If Simulink 3D Animation is available, the visualization will also include a planar checkerboard surface (changing the default scene may be desired in the Visualization subsystem).
      mask init:
      | vehdynicon('vehdynlibzplane',gcb,0,[]);
      mask Callback plane3D: vehdynicon('vehdynlibzplane',gcb,1,[]);
      mask DialogControl initParams Prompt: Setup Parameters
      mask DialogControl slddUpdate Prompt: Vehicle Pose Estimates
      mask DialogControl updateSLDD Prompt: Update data dictionary with initial roll, pitch and yaw estimates
      mask DialogControl updateSLDD Callback: vehdynicon('vehdynlibzplane',gcb,2,'VirtualVehicleTemplate.sldd');
      mask DialogControl sim3d Prompt: Visualization Options
  Rate Limiter : RateLimiter  RisingSlewLimit=10  FallingSlewLimit=-10  SampleTimeMode=inherited
  Rate Limiter1 : RateLimiter  RisingSlewLimit=10  FallingSlewLimit=-10  SampleTimeMode=inherited
  Signal Specification : SignalSpecification  Unit=m
  Signal Specification1 : SignalSpecification  Unit=deg
  Signal Specification2 : SignalSpecification  Unit=deg
  Slider : SliderBlock  ScaleMin=-30  ScaleMax=30
  Slider1 : SliderBlock  ScaleMin=-30  ScaleMax=30
  Unit Conversion : UnitConversion
  Unit Conversion1 : UnitConversion
  Vector Concatenate : Concatenate  NumInputs=4  Mode=Multidimensional array  ConcatenateDimension=3
  Wheel Coordinates : Subsystem
  Z+up : UnaryMinus
  phiPlane : Constant  Value=0
  thetaPlane : Constant  Value=0
  Z : Outport
  DCM : Outport  Port=2
  wires:
  Ideal Inclined Plane/2(DCM) -> Vector Concatenate/1, Vector Concatenate/2, Vector Concatenate/4, Vector Concatenate/3  "DCM"
  Signal Specification/1 -> Demux/1
  Bus Creator/1 -> Z/1  "z"
  Demux/3 -> Bus Creator/3  "G_RL_z"
  Demux/4 -> Bus Creator/4  "G_RR_z"
  Demux/1 -> Bus Creator/1  "G_FL_z"
  Demux/2 -> Bus Creator/2  "G_FR_z"
  InertFrm/1 -> Bus Selector/1, Bus Selector1/1
  Wheel Coordinates/1(XWhl) -> Ideal Inclined Plane/1(X)
  Wheel Coordinates/2(YWhl) -> Z+up/1
  Bus Selector1/1 -> Wheel Coordinates/5(FrntAxlLftY)  "<Y>"
  Bus Selector/3 -> Wheel Coordinates/3(RearAxlLftX)  "<X>"
  Bus Selector/4 -> Wheel Coordinates/4(RearAxlRghtX)  "<X>"
  Bus Selector1/2 -> Wheel Coordinates/6(FrntAxlRghtY)  "<Y>"
  Bus Selector/2 -> Wheel Coordinates/2(FrntAxlRghtX)  "<X>"
  Bus Selector/1 -> Wheel Coordinates/1(FrntAxlLftX)  "<X>"
  Bus Selector1/3 -> Wheel Coordinates/7(RearAxlLftY)  "<Y>"
  Bus Selector1/4 -> Wheel Coordinates/8(RearAxlRghtY)  "<Y>"
  phiPlane/1 -> Rate Limiter/1
  Ideal Inclined Plane/1(Z) -> Signal Specification/1
  thetaPlane/1 -> Rate Limiter1/1
  Z+up/1 -> Ideal Inclined Plane/2(Y)
  Signal Specification2/1 -> Unit Conversion1/1
  Signal Specification1/1 -> Unit Conversion/1
  Unit Conversion1/1 -> Ideal Inclined Plane/3(phi)
  Unit Conversion/1 -> Ideal Inclined Plane/4(theta)
  Vector Concatenate/1 -> DCM/1  "DCM"
  Rate Limiter/1 -> Signal Specification2/1
  Rate Limiter1/1 -> Signal Specification1/1

== system ConfiguredHevMmVirtualVehicle/Environment/Ground Feedback/Three-Axle Constant ==
  Bus Creator : BusCreator  Inputs=6
  Constant1 : Constant  Value=zeros(6,1)
  Constant2 : Constant  Value=repmat(eye(3),1,1,6)  SampleTime=-1
  Demux : Demux  Outputs=6
  Signal Specification : SignalSpecification  Unit=m
  Z : Outport  VectorParamsAs1DForOutWhenUnconnected=off
  DCM : Outport  Port=2  VectorParamsAs1DForOutWhenUnconnected=off
  wires:
  Demux/4 -> Bus Creator/4  "G_MR_z"
  Constant2/1 -> DCM/1  "DCM"
  Bus Creator/1 -> Z/1  "z"
  Demux/2 -> Bus Creator/2  "G_FR_z"
  Demux/3 -> Bus Creator/3  "G_ML_z"
  Signal Specification/1 -> Demux/1
  Constant1/1 -> Signal Specification/1
  Demux/6 -> Bus Creator/6  "G_RR_z"
  Demux/5 -> Bus Creator/5  "G_RL_z"
  Demux/1 -> Bus Creator/1  "G_FL_z"

== system ConfiguredHevMmVirtualVehicle/Environment/Subsystem/Estimated Grade ==
  Gnd : Inport
  Atan : Trigonometry  Operator=atan
  Bus Selector : BusSelector  OutputSignals=z  OutputAsBus=on
  Bus to Vector : BusToVector
  Constant Grade : Constant  Value=EnvNominalGrade  SampleTime=-1
  Constant1 : Constant  Value=PlntVehDstCGFrntAxl+PlntVehDstCGRearAxl  SampleTime=-1
  Divide : Product  Inputs=*/
  Gain : Gain  Gain=.5
  Gain1 : Gain  Gain=.5
  Grade Source : ManualSwitch  CurrentSetting=0
  Signal Specification : SignalSpecification  Unit=rad
  Signal Specification1 : SignalSpecification  Unit=deg
  Signal Specification2 : SignalSpecification  Unit=deg
  Subtract : Sum  Inputs=+-
  Sum of Elements : Sum  Inputs=+
  Sum of Elements1 : Sum  Inputs=+
  Unit Conversion : UnitConversion
  Variant Subsystem : Subsystem  Variant=on  VariantControlMode=label  LabelModeActiveChoice=TwoAxle
  Grade : Outport  PortDimensions=1
  wires:
  Divide/1 -> Atan/1
  Bus Selector/1 -> Bus to Vector/1
  Sum of Elements/1 -> Gain/1
  Gain/1 -> Subtract/1
  Sum of Elements1/1 -> Gain1/1
  Signal Specification/1 -> Unit Conversion/1
  Constant1/1 -> Divide/2
  Gain1/1 -> Subtract/2
  Subtract/1 -> Divide/1
  Atan/1 -> Signal Specification/1
  Grade Source/1 -> Grade/1  "Grade"
  Gnd/1 -> Bus Selector/1
  Bus to Vector/1 -> Variant Subsystem/1(Gnd)
  Constant Grade/1 -> Signal Specification2/1
  Signal Specification2/1 -> Grade Source/2
  Unit Conversion/1 -> Signal Specification1/1
  Signal Specification1/1 -> Grade Source/1  "Grade"
  Variant Subsystem/1(F) -> Sum of Elements/1
  Variant Subsystem/2(R) -> Sum of Elements1/1

== system ConfiguredHevMmVirtualVehicle/Environment/Subsystem/Variant Subsystem ==
  note: 1) Add Subsystem or Model blocks as valid variant choices.
      | 2) You cannot connect blocks at this level. At simulation, connectivity is automatically
      | determined, based on the active variant and port name matching.
  InGnd : Inport
  Three-Axle : Subsystem  VariantControl=ThreeAxle
  Two-Axle : Subsystem  VariantControl=TwoAxle
  z : Outport
  <DCM> : Outport  Port=2
  lambda_mux : Outport  Port=3

== system ConfiguredHevMmVirtualVehicle/Environment/Varying Friction/Constant Friction ==
  Friction Scaling : Constant  Value=ones(4,1).*EnvNomFrictionScaling  SampleTime=0
  FricCoeffLambda : Outport
  wires:
  Friction Scaling/1 -> FricCoeffLambda/1

== system ConfiguredHevMmVirtualVehicle/Environment/Varying Friction/Friction Map ==
  InertFrm : Inport
  2D Lookup Tbl for Scaling Fctr (Lambda) : Subsystem  TreatAsAtomicUnit=on
      mask init:
      | [~]=vehdynicon('vehdynblk',gcb);
  Bus Selector : BusSelector  OutputSignals=FrntAxl.Lft.Disp.X,FrntAxl.Rght.Disp.X,RearAxl.Lft.Disp.X,RearAxl.Rght.Disp.X
  Bus Selector1 : BusSelector  OutputSignals=FrntAxl.Lft.Disp.Y,FrntAxl.Rght.Disp.Y,RearAxl.Lft.Disp.Y,RearAxl.Rght.Disp.Y
  Wheel Coordinates : Subsystem
  FricCoeffLambda : Outport
  wires:
  InertFrm/1 -> Bus Selector1/1, Bus Selector/1
  2D Lookup Tbl for Scaling Fctr (Lambda)/1(FricCoeffLambda) -> FricCoeffLambda/1
  Bus Selector1/4 -> Wheel Coordinates/8(RearAxlRghtY)  "<Y>"
  Bus Selector1/3 -> Wheel Coordinates/7(RearAxlLftY)  "<Y>"
  Bus Selector/1 -> Wheel Coordinates/1(FrntAxlLftX)  "<X>"
  Bus Selector/2 -> Wheel Coordinates/2(FrntAxlRghtX)  "<X>"
  Bus Selector1/2 -> Wheel Coordinates/6(FrntAxlRghtY)  "<Y>"
  Bus Selector/4 -> Wheel Coordinates/4(RearAxlRghtX)  "<X>"
  Bus Selector/3 -> Wheel Coordinates/3(RearAxlLftX)  "<X>"
  Bus Selector1/1 -> Wheel Coordinates/5(FrntAxlLftY)  "<Y>"
  Wheel Coordinates/2(YWhl) -> 2D Lookup Tbl for Scaling Fctr (Lambda)/2(YWhl)
  Wheel Coordinates/1(XWhl) -> 2D Lookup Tbl for Scaling Fctr (Lambda)/1(XWhl)

== system ConfiguredHevMmVirtualVehicle/Environment/Varying Friction/Three-Axle Constant Friction ==
  Friction Scaling : Constant  Value=ones(6,1).*EnvNomFrictionScaling  SampleTime=0
  FricCoeffLambda : Outport
  wires:
  Friction Scaling/1 -> FricCoeffLambda/1

== system ConfiguredHevMmVirtualVehicle/Environment/Varying Friction/Varying Friction ==
  InertFrm : Inport
  Cg : Inport  Port=2
  Bus Selector : BusSelector  OutputSignals=FrntAxl.Lft.Disp.X,FrntAxl.Rght.Disp.X,RearAxl.Lft.Disp.X,RearAxl.Rght.Disp.X
  Bus Selector1 : BusSelector  OutputSignals=FrntAxl.Lft.Disp.Y,FrntAxl.Rght.Disp.Y,RearAxl.Lft.Disp.Y,RearAxl.Rght.Disp.Y
  Road Track Friction : Subsystem  mask(Road Track Friction){surface_popup=Split friction coefficient scaling factor, lambda_g=EnvNomFrictionScaling, lambda_r=.6, r_x0=175, r_y0=-100, r_xw=1000, r_yw=500, aMode=2}
      mask prompts: surface_popup "Type of surface:"; lambda_g "Scaling factor for the friction coefficient of ground, lambda_g :"; lambda_r "Scaling factor for the friction coefficient of rectangular surface, lambda_r :"; r_x0 "X coordinate of lower left corner of rectangular surface, r_x0 [m]:"; r_y0 "Y coordinate of lower left corner of rectangular surface, r_y0 [m]:"; r_xw "Rectangular surface width in X direction, r_xw [m]:"; r_yw "Rectangular surface width in Y direction, r_yw [m]:"
      mask init:
      | % Scaling factor for the friction coefficient around the rectangular region
      | mutable = [lambda_g, lambda_g, lambda_g, lambda_g;
      |            lambda_g, lambda_r, lambda_r, lambda_g; 
      |            lambda_g, lambda_r, lambda_r, lambda_g; 
      |            lambda_g, lambda_g, lambda_g, lambda_g ];
      |        
      | 
      | % The step is distance between breakpoint near the boundary of high and
      | % low friction coefficient
      | 
      | step = 0.01 ; 
      | 
      | % In the mask initialization, xbr and ybr breakpoints are with respect to
      | % Body fixed coordinate system. At time t=0, xbr and ybr breakpoints
      | % updates to Earth (Inertial) Fixed coordinate system. The breakpoints for
      | % the lookup table are added via inputs.
      | 
      | xbr = [(r_x0 - step) , (r_x0 + step), (r_x0 + r_xw - step) , (r_x0 + r_xw + step) ];
      | ybr = [(r_y0 - step) , (r_y0 + step), (r_y0 + r_yw - step) , (r_y0 + r_yw + step) ];
      | 
      | 
      | % To check if the created track is split mu or constant mu
      | 
      | surface_popup = get_param(gcb, 'surface_popup');
      | 
      | if strcmp(surface_popup, 'Split friction coefficient scaling factor')
      |     SplitLambdaTrck = 1;
      | elseif strcmp(surface_popup, 'Constant friction coefficient scaling factor')
      |     SplitLambdaTrck = 0;
      | end
      mask Help: eval('vdynblkshelp(''vdynblkstrack'')');
      mask TypeOptions surface_popup: Constant friction coefficient scaling factor | Split friction coefficient scaling factor
      mask Callback surface_popup:
      | surface_popup = get_param(gcb, 'surface_popup');
      | m = Simulink.Mask.get(gcb);
      | 
      | lambda_g = m.getParameter('lambda_g');
      | lambda_r = m.getParameter('lambda_r');
      | r_x0 = m.getParameter('r_x0');
      | r_y0 = m.getParameter('r_y0');
      | r_xw = m.getParameter('r_xw');
      | r_yw = m.getParameter('r_yw');
      | %track_view = m.getParameter('track_view');
      | 
      | 
      | if strcmp(surface_popup, 'Split friction coefficient scaling factor')
      |     lambda_g.Visible = 'on';
      |     lambda_r.Visible = 'on';
      |     r_x0.Visible = 'on';
      |     r_y0.Visible = 'on';
      |     r_xw.Visible = 'on';
      |     r_yw.Visible = 'on';
      |     %track_view.Visible = 'on';
      | 
      | elseif strcmp(surface_popup,'Constant friction coefficient scaling factor')
      |     lambda_g.Visible = 'on';
      |     lambda_r.Visible = 'off';
      |     r_x0.Visible = 'off';
      |     r_y0.Visible = 'off';
      |     r_xw.Visible = 'off';
      |     r_yw.Visible = 'off';
      |     %track_view.Visible = 'off';
      | end
      | [~]=autosharedicon('autolibutils',gcb,0);
      mask DialogControl DescGroupVar Prompt: Track description  (mask)
      mask DialogControl DescTextVar Prompt: Generates a default or user-specified track which creates a rectangular surface of specified friction coefficient. The location of rectangular surface is relative to the origin of Body Fixed Coordinate System.The input of the block is X and Y coordinates of the wheel from the vehicle feedback bus. The block output is friction coefficient for all the wheels.
  Wheel Coordinates : Subsystem
  FricCoeffLambda : Outport
  wires:
  Bus Selector1/1 -> Wheel Coordinates/5(FrntAxlLftY)  "<Y>"
  Bus Selector/3 -> Wheel Coordinates/3(RearAxlLftX)  "<X>"
  Bus Selector/4 -> Wheel Coordinates/4(RearAxlRghtX)  "<X>"
  Wheel Coordinates/1(XWhl) -> Road Track Friction/1(XWhl)
  Bus Selector1/2 -> Wheel Coordinates/6(FrntAxlRghtY)  "<Y>"
  Bus Selector/2 -> Wheel Coordinates/2(FrntAxlRghtX)  "<X>"
  Bus Selector/1 -> Wheel Coordinates/1(FrntAxlLftX)  "<X>"
  Bus Selector1/3 -> Wheel Coordinates/7(RearAxlLftY)  "<Y>"
  Bus Selector1/4 -> Wheel Coordinates/8(RearAxlRghtY)  "<Y>"
  Cg/1 -> Road Track Friction/3(Cg)
  Wheel Coordinates/2(YWhl) -> Road Track Friction/2(YWhl)
  Road Track Friction/1(FricCoeffLambda) -> FricCoeffLambda/1
  InertFrm/1 -> Bus Selector1/1, Bus Selector/1

== system ConfiguredHevMmVirtualVehicle/Scenarios/Coordinate Systems/ISO 8855 (Z-up) ==
  ExtDrvRefIn : Inport
  ExtDrvCmdIn : Inport  Port=2
  Bus Assignment : BusAssignment  AssignedSignals=LtrRef,YRef,PhiRef,CurvRef,CurvGradRef
  Bus Assignment1 : BusAssignment  AssignedSignals=SteerCmd.SteerCmd
  Bus Selector : BusSelector  OutputSignals=LtrRef,YRef,PhiRef,CurvRef,CurvGradRef
  Bus Selector1 : BusSelector  OutputSignals=SteerCmd.SteerCmd
  Unary Minus{,1..5} (6 alike) : UnaryMinus
  ExtDrvRef : Outport
  ExtDrvCmd : Outport  Port=2
  wires:
  ExtDrvRefIn/1 -> Bus Assignment/1, Bus Selector/1
  ExtDrvCmdIn/1 -> Bus Assignment1/1, Bus Selector1/1
  Unary Minus/1 -> Bus Assignment/2
  Bus Assignment1/1 -> ExtDrvCmd/1
  Bus Assignment/1 -> ExtDrvRef/1
  Bus Selector/1 -> Unary Minus/1  "<LtrRef>"
  Unary Minus2/1 -> Bus Assignment/3
  Unary Minus3/1 -> Bus Assignment/4
  Unary Minus4/1 -> Bus Assignment/5
  Unary Minus5/1 -> Bus Assignment/6
  Bus Selector/2 -> Unary Minus2/1  "<YRef>"
  Bus Selector/3 -> Unary Minus3/1  "<PhiRef>"
  Bus Selector/4 -> Unary Minus4/1  "<CurvRef>"
  Bus Selector/5 -> Unary Minus5/1  "<CurvGradRef>"
  Unary Minus1/1 -> Bus Assignment1/2
  Bus Selector1/1 -> Unary Minus1/1  "<SteerCmd>"

== system ConfiguredHevMmVirtualVehicle/Scenarios/Coordinate Systems/SAE J670 (Z-down) ==
  ExtDrvRefIn : Inport
  ExtDrvCmdIn : Inport  Port=2
  ExtDrvRef : Outport
  ExtDrvCmd : Outport  Port=2
  wires:
  ExtDrvCmdIn/1 -> ExtDrvCmd/1
  ExtDrvRefIn/1 -> ExtDrvRef/1

== system ConfiguredHevMmVirtualVehicle/Scenarios/Reference Generator/Braking ==
  "VehFdbk " : Inport
  Braking : vehdynlibscenariocommon/Acceleration and Deceleration Signal Input  tStart=ScnStartTime  ax=ScnBrkAx  velRef=ScnLongVelRef  velRefUnit=mph  brakingType=Longitudinal displacement  tBrake=15  xBrake=ScnBrkXbrake  axDecel=ScnBrkAxdec  steerZero=on  faultTracking=off  bufferSize=4096  velMaxDiff=1  velMeanDiff=2  rMaxDiff=1  steerMaxDiff=3  stopOnFault=off  aMode=2
      settings: LibrarySourceBlock=vehdynlibscenario/Acceleration and Braking
  Bus Creator : BusCreator  Inputs=3
  Bus Selector : BusSelector  OutputSignals=Body.BdyFrm.Cg.Vel.xdot
  Constant : Constant  Value=0
  Constant1 : Constant  Value=0
  Constant2 : Constant  Value=0
  " Vis" : Outport
  DrvRef : Outport  Port=2  VectorParamsAs1DForOutWhenUnconnected=off
  DrvCmd : Outport  Port=3  VectorParamsAs1DForOutWhenUnconnected=off
  " Fdbk" : Outport  Port=4  VectorParamsAs1DForOutWhenUnconnected=off
  wires:
  "VehFdbk "/1 -> " Fdbk"/1, Bus Selector/1
  Braking/2 -> DrvCmd/1
  Bus Selector/1 -> Braking/1  "<xdot>"
  Braking/1 -> DrvRef/1
  Constant/1 -> Bus Creator/1  "XRef"
  Constant1/1 -> Bus Creator/2  "YRef"
  Bus Creator/1 -> " Vis"/1
  Constant2/1 -> Bus Creator/3  "ZRef"
